simulink model "ex2"  (R2025b)
settings: Solver=FixedStepAuto  StartTime=0.0  StopTime=0.16  FixedStep=1e-5  RelTol=1e-4
values from neighbouring files (symbols this model uses):
  In = 20    [sim1.m]
  J = 0.001    [sim1.m]
  ki = ac^2*L    [sim1.m]
  kp = ac*L    [sim1.m]
  L = 2.5e-3    (= 0.0025)    [sim1.m]
  psi = 0.35    [sim1.m]
  R = 0.5    [sim1.m]
  Ra = ac*L-R    [sim1.m]
  Vn = 120    [sim1.m]
  wn = Nn*2*pi/60    (= 314.159265359)    [sim1.m]
settings Model: Creator=dimit  LastModifiedBy=Dimitris

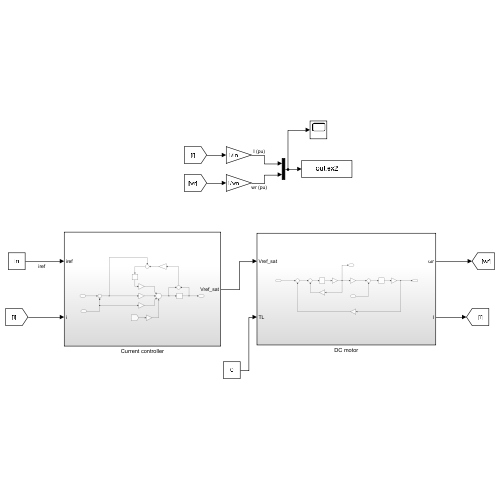
[thumbnail: Simulink's stored preview of the top-level diagram]
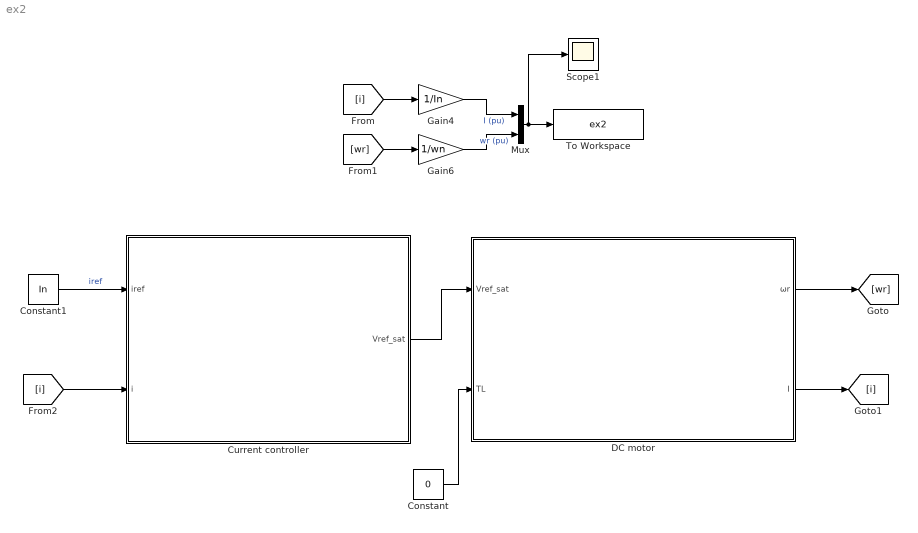
== system ex2 ==
  Constant : Constant  Value=0
  Constant1 : Constant  Value=In
  Current controller : Subsystem
  DC motor : Subsystem
  Gain4 : Gain  Gain=1/In
  Gain6 : Gain  Gain=1/wn
  Mux : Mux  Inputs=2
  Scope1 : Scope
      settings: ActiveDisplayYMinimum=-0.37012928995988681  ActiveDisplayYMaximum=1.2935533510809303
  To Workspace : ToWorkspace  VariableName=ex2  SaveFormat=Timeseries  SampleTime=-1
  wires:
  Current controller/1(Vref_sat) -> DC motor/1(Vref_sat)
  Constant1/1 -> Current controller/1(iref)  "iref"
  [i] -> Current controller/2(i)
  DC motor/1(ωr) -> [wr]
  Gain4/1 -> Mux/1  "I (pu)"
  [i] -> Gain4/1
  Mux/1 -> Scope1/1, To Workspace/1
  Gain6/1 -> Mux/2  "wr (pu)"
  [wr] -> Gain6/1
  Constant/1 -> DC motor/2(TL)
  DC motor/2(I) -> [i]

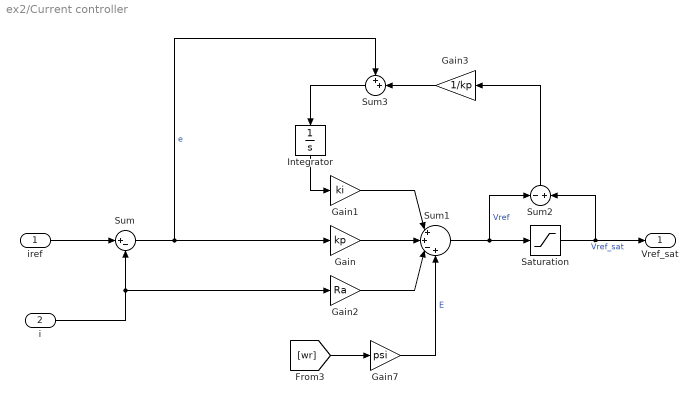
== system ex2/Current controller ==
  iref : Inport
  i : Inport  Port=2
  Gain : Gain  Gain=kp
  Gain1 : Gain  Gain=ki
  Gain2 : Gain  Gain=Ra
  Gain3 : Gain  Gain=1/kp
  Gain7 : Gain  Gain=psi
  Integrator : Integrator
  Saturation : Saturate  UpperLimit=Vn  LowerLimit=-Vn
  Sum : Sum  Inputs=|+-
  Sum1 : Sum  Inputs=|++-+
  Sum2 : Sum  Inputs=-|+
  Sum3 : Sum  Inputs=++|
  Vref_sat : Outport
  wires:
  Saturation/1 -> Vref_sat/1, Sum2/2  "Vref_sat"
  Sum2/1 -> Gain3/1
  Gain7/1 -> Sum1/4  "E"
  [wr] -> Gain7/1
  Gain3/1 -> Sum3/2
  Sum1/1 -> Sum2/1, Saturation/1  "Vref"
  Gain/1 -> Sum1/2
  Sum3/1 -> Integrator/1
  i/1 -> Sum/2, Gain2/1
  Sum/1 -> Sum3/1, Gain/1  "e"
  Gain2/1 -> Sum1/3
  Gain1/1 -> Sum1/1
  iref/1 -> Sum/1
  Integrator/1 -> Gain1/1

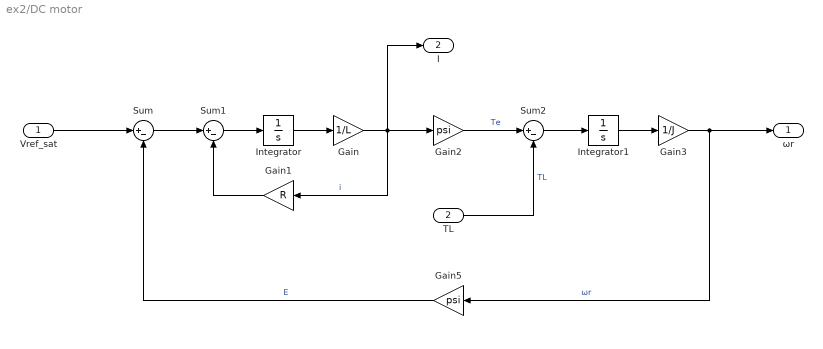
== system ex2/DC motor ==
  Vref_sat : Inport
  TL : Inport  Port=2
  Gain : Gain  Gain=1/L
  Gain1 : Gain  Gain=R
  Gain2 : Gain  Gain=psi
  Gain3 : Gain  Gain=1/J
  Gain5 : Gain  Gain=psi
  Integrator : Integrator
  Integrator1 : Integrator
  Sum : Sum  Inputs=|+-
  Sum1 : Sum  Inputs=|+-
  Sum2 : Sum  Inputs=|+-
  ωr : Outport
  I : Outport  Port=2
  wires:
  Gain/1 -> I/1, Gain2/1, Gain1/1  "i"
  Gain2/1 -> Sum2/1  "Te"
  Sum/1 -> Sum1/1
  Integrator1/1 -> Gain3/1
  Integrator/1 -> Gain/1
  Gain3/1 -> ωr/1, Gain5/1  "ωr"
  Sum2/1 -> Integrator1/1
  TL/1 -> Sum2/2  "TL"
  Gain5/1 -> Sum/2  "E"
  Gain1/1 -> Sum1/2
  Sum1/1 -> Integrator/1
  Vref_sat/1 -> Sum/1
